simulink model "DC_control"  (R2023b)
settings: Solver=ode45  StartTime=0.0  StopTime=700  RelTol=1e-3
values from neighbouring files (symbols this model uses):
  g = 9.81    [Parameters_estimation.m]
  Ia_n = (Ptot-Ve_n*Ie_n)/Va_n    [Parameters_estimation.m]    (also in psi_ref_parameters.mat = 650.546469803)
  Ke = Pn/(Ie_n*Ia_n*w_n)    [Parameters_estimation.m]    (also in psi_ref_parameters.mat = 1.72027393081)
  M = 10*10^3+80*200    (= 26000)    [Parameters_estimation.m]
  mu_Ia = 1/Ra    [Parameters_estimation.m]
  mu_Ie = 1/Re    (= 0.00833333333333)    [Parameters_estimation.m]
  mu_m = 1/(R^2*betha)    [Parameters_estimation.m]
  R = v_n/w_n    (= 0.0530785562633)    [Parameters_estimation.m]    (also in Radius.mat; my_parameters.mat)
  T_n = Ft_n * R    [Parameters_estimation.m]
  tau_Ia = La/Ra    [Parameters_estimation.m]
  tau_Ie = Le/Re    (= 1)    [Parameters_estimation.m]
  tau_m = M/betha    [Parameters_estimation.m]
  Va_n = 600    [Parameters_estimation.m]    (also in psi_ref_parameters.mat)
  Ve_n = 120    [Parameters_estimation.m]
  wc_Ia = 100    [Parameters_estimation.m]
  wc_Ie = 10    [Parameters_estimation.m]
  wc_ome = 5/(t_fin-20)    (= 1)    [Parameters_estimation.m]
libraries: slpidlib x3
settings Model: Creator=lmarz  LastModifiedBy=lmarz

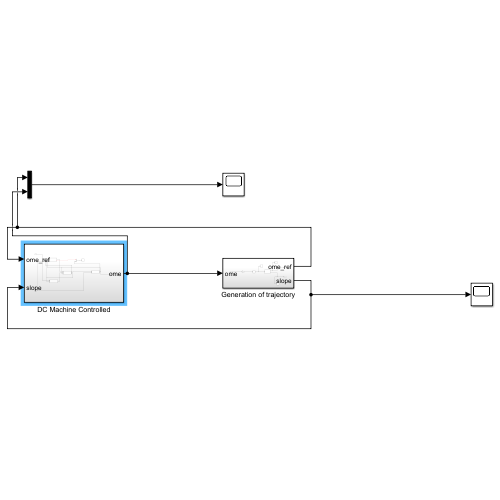
[thumbnail: Simulink's stored preview of the top-level diagram]
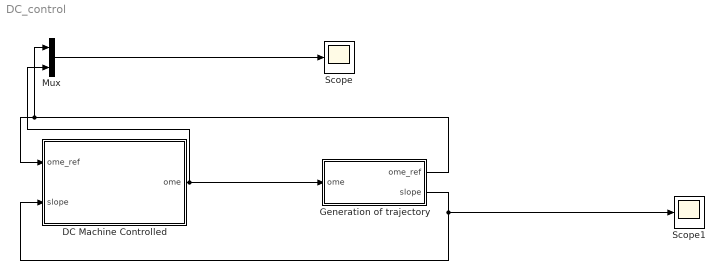
== system DC_control ==
  DC Machine Controlled : Subsystem
  Generation of trajectory : Subsystem
  Mux : Mux  Inputs=2
  Scope : Scope
  Scope1 : Scope
  wires:
  DC Machine Controlled/1(ome) -> Mux/2, Generation of trajectory/1(ome)
  Generation of trajectory/1(ome_ref) -> Mux/1, DC Machine Controlled/1(ome_ref)
  Generation of trajectory/2(slope) -> Scope1/1, DC Machine Controlled/2(slope)
  Mux/1 -> Scope/1

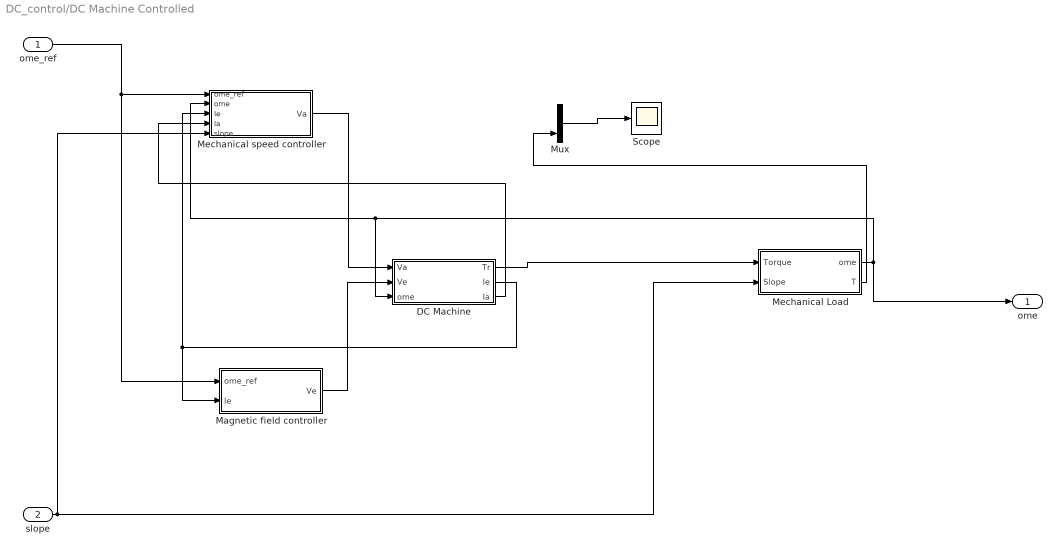
== system DC_control/DC Machine Controlled ==
  ome_ref : Inport
  slope : Inport  Port=2
  " Mechanical speed controller" : Subsystem
  DC Machine : Subsystem
  Magnetic field controller : Subsystem
  Mechanical Load : Subsystem
  Mux : Mux  Inputs=2
  Scope : Scope
  ome : Outport
  wires:
  DC Machine/1(Tr) -> Mechanical Load/1(Torque)
  Mechanical Load/1(ome) -> ome/1, DC Machine/3(ome), " Mechanical speed controller"/2(ome)
  ome_ref/1 -> Magnetic field controller/1(ome_ref), " Mechanical speed controller"/1(ome_ref)
  Magnetic field controller/1(Ve) -> DC Machine/2(Ve)
  DC Machine/2(Ie) -> " Mechanical speed controller"/3(Ie), Magnetic field controller/2(Ie)
  DC Machine/3(Ia) -> " Mechanical speed controller"/4(Ia)
  " Mechanical speed controller"/1(Va) -> DC Machine/1(Va)
  slope/1 -> " Mechanical speed controller"/5(slope), Mechanical Load/2(Slope)
  ? -> Mux/1
  Mechanical Load/2(T) -> Mux/2
  Mux/1 -> Scope/1

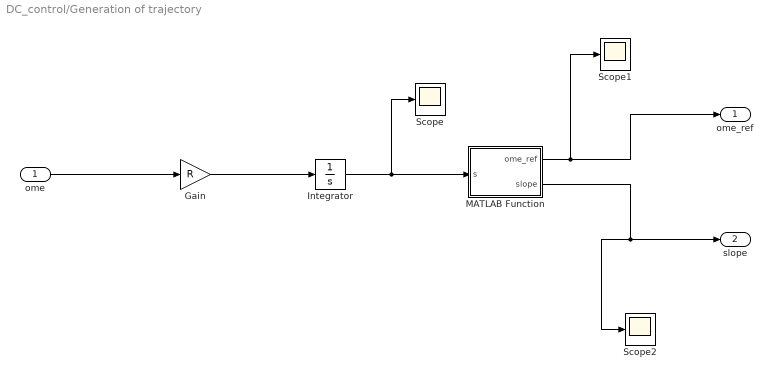
== system DC_control/Generation of trajectory ==
  ome : Inport
  Gain : Gain  Gain=R
  Integrator : Integrator
  MATLAB Function : MATLAB Function  TreatAsAtomicUnit=on
  Scope : Scope
  Scope1 : Scope
  Scope2 : Scope
  ome_ref : Outport
  slope : Outport  Port=2
  wires:
  ome/1 -> Gain/1
  Gain/1 -> Integrator/1
  Integrator/1 -> Scope/1, MATLAB Function/1(s)
  MATLAB Function/1(ome_ref) -> Scope1/1, ome_ref/1
  MATLAB Function/2(slope) -> Scope2/1, slope/1

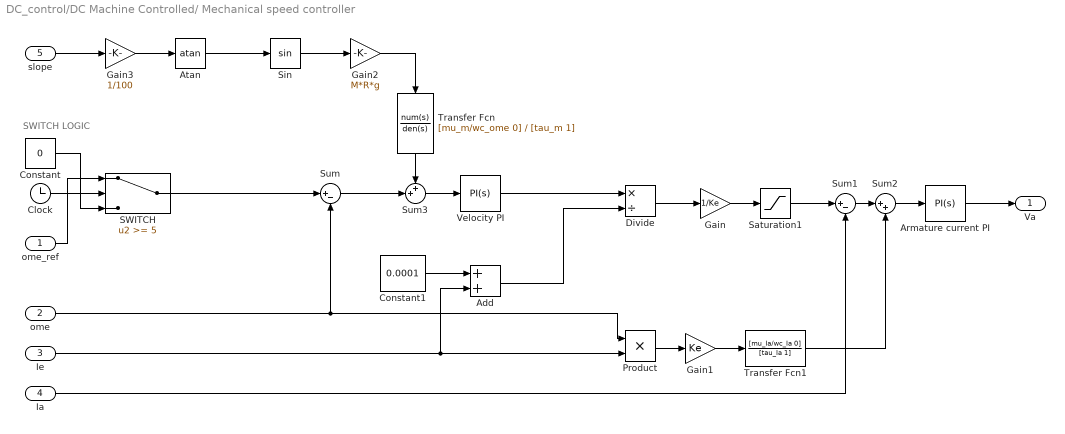
== system DC_control/DC Machine Controlled/ Mechanical speed controller ==
  note: SWITCH LOGIC
  ome_ref : Inport
  ome : Inport  Port=2
  Ie : Inport  Port=3
  Ia : Inport  Port=4
  slope : Inport  Port=5
  Add : Sum
  Armature current PI : slpidlib/PID Controller  Controller=PI  Form=Parallel  TimeDomain=Continuous-time  UseExternalTs=off  SampleTime=-1  IntegratorMethod=Forward Euler  FilterMethod=Forward Euler  ControllerParametersSource=internal  P=wc_Ia*tau_Ia/mu_Ia  I=wc_Ia/mu_Ia  UseKiTs=off  D=0  N=100  UseFilter=on  TunerSelectOption=Transfer Function Based (PID Tuner App)  ZeroCross=off  InitialConditionSource=internal  InitialConditionForIntegrator=0  InitialConditionForFilter=0  DifferentiatorICPrevScaledInput=0  ExternalReset=none  TrackingMode=off  Kt=1  LimitOutput=on  SatLimitsSource=internal  UpperSaturationLimit=Va_n  LowerSaturationLimit=-Va_n  LinearizeAsGain=on  AntiWindupMode=clamping  Kb=1  LimitIntegrator=off  UpperIntegratorSaturationLimit=inf  LowerIntegratorSaturationLimit=-inf  POutMin=[]  POutMax=[]  IOutMin=[]  IOutMax=[]  DOutMin=[]  DOutMax=[]  NOutMin=[]  NOutMax=[]  SumOutMin=[]  SumOutMax=[]  SaturationOutMin=[]  SaturationOutMax=[]  PParamMin=[]  PParamMax=[]  IParamMin=[]  IParamMax=[]  DParamMin=[]  DParamMax=[]  NParamMin=[]  NParamMax=[]  KbParamMin=[]  KbParamMax=[]  KtParamMin=[]  KtParamMax=[]  KbOutMin=[]  KbOutMax=[]  KtOutMin=[]  KtOutMax=[]  IntegratorOutMin=[]  IntegratorOutMax=[]  FilterOutMin=[]  FilterOutMax=[]  SumI1OutMin=[]  SumI1OutMax=[]  SumI2OutMin=[]  SumI2OutMax=[]  SumI3OutMin=[]  SumI3OutMax=[]  SumI4OutMin=[]  SumI4OutMax=[]  SumDOutMin=[]  SumDOutMax=[]  DifferentiatorOutMin=[]  DifferentiatorOutMax=[]  FilterDiffOutCoefMin=[]  FilterDiffOutCoefMax=[]  ReciprocalOutMin=[]  ReciprocalOutMax=[]  SumDenOutMin=[]  SumDenOutMax=[]  SumNumOutMin=[]  SumNumOutMax=[]  DivideOutMin=[]  DivideOutMax=[]  UdiffTsProdOutMin=[]  UdiffTsProdOutMax=[]  NTsProdOutMin=[]  NTsProdOutMax=[]  UintegralTsProdOutMin=[]  UintegralTsProdOutMax=[]  UngainTsProdOutMin=[]  UngainTsProdOutMax=[]  ClampingZeroOutDataTypeStr=Inherit: Inherit via back propagation  ClampingZeroOutMin=[]  ClampingZeroOutMax=[]  FilterDenConstantOutDataTypeStr=Inherit: Inherit via back propagation  FilterDenConstantOutMin=[]  FilterDenConstantOutMax=[]  PCopyOutDataTypeStr=Inherit: Inherit via back propagation  PCopyOutMin=[]  PCopyOutMax=[]  NCopyOutDataTypeStr=Inherit: Inherit via back propagation  NCopyOutMin=[]  NCopyOutMax=[]  IntegratorContinuousStateAttributes=''  IntegratorStateMustResolveToSignalObject=off  IntegratorRTWStateStorageClass=Auto  FilterContinuousStateAttributes=''  FilterStateMustResolveToSignalObject=off  FilterRTWStateStorageClass=Auto  ParallelPVariant=InternalParameters  IdealPVariant=Disabled  IVariant=InternalParameters  DVariant=Disabled  IntegratorVariant=Continuous  SatVariant=Enabled  AWVariant=ContClampingParallel  PCopyVariant=Disabled  TRVariant=Disabled  FdbkBlocksVariant=Forward  IdealPFdbkVariant=Disabled  SatFdbkVariant=Disabled  DerivativeFilterVariant=Disabled  NVariant=Disabled  NCopyVariant=Disabled_SignalSpec  FilterICVariant=Disabled  IntegratorICVariant=InternalICs  ExternalResetVariant=Disabled  TRSumVariant=Passthrough  SumFdbkVariant=Disabled  SumVariant=Sum_PI  TsampFilterVariant=InternalTs  TsampNgainVariant=Passthrough  TsampIntegralVariant=Disabled_SignalSpec  ExternalSaturationOutDataTypeStr=Inherit: Same as second input
  Atan : Trigonometry  Operator=atan
  Clock : Clock
  Constant : Constant  Value=0
  Constant1 : Constant  Value=0.0001
  Divide : Product  Inputs=*/
  Gain : Gain  Gain=1/Ke
  Gain1 : Gain  Gain=Ke
  Gain2 : Gain  Gain=M*R*g
  Gain3 : Gain  Gain=1/100
  Product : Product
  SWITCH : Switch  Threshold=5  SaturateOnIntegerOverflow=off  InputSameDT=off
  Saturation1 : Saturate  UpperLimit=Ia_n  LowerLimit=-Ia_n
  Sin : Trigonometry
  Sum : Sum  Inputs=|+-
  Sum1 : Sum  Inputs=|+-
  Sum2 : Sum  Inputs=|++
  Sum3 : Sum  Inputs=++|
  Transfer Fcn : TransferFcn  Numerator=[mu_m/wc_ome 0]  Denominator=[tau_m 1]
  Transfer Fcn1 : TransferFcn  Numerator=[mu_Ia/wc_Ia 0]  Denominator=[tau_Ia 1]
  Velocity PI : slpidlib/PID Controller  Controller=PI  Form=Parallel  TimeDomain=Continuous-time  UseExternalTs=off  SampleTime=-1  IntegratorMethod=Forward Euler  FilterMethod=Forward Euler  ControllerParametersSource=internal  P=wc_ome*tau_m/mu_m  I=wc_ome/mu_m  UseKiTs=off  D=0  N=100  UseFilter=on  TunerSelectOption=Transfer Function Based (PID Tuner App)  ZeroCross=off  InitialConditionSource=internal  InitialConditionForIntegrator=0  InitialConditionForFilter=0  DifferentiatorICPrevScaledInput=0  ExternalReset=none  TrackingMode=off  Kt=1  LimitOutput=on  SatLimitsSource=internal  UpperSaturationLimit=T_n  LowerSaturationLimit=-T_n  LinearizeAsGain=on  AntiWindupMode=clamping  Kb=1  LimitIntegrator=off  UpperIntegratorSaturationLimit=inf  LowerIntegratorSaturationLimit=-inf  POutMin=[]  POutMax=[]  IOutMin=[]  IOutMax=[]  DOutMin=[]  DOutMax=[]  NOutMin=[]  NOutMax=[]  SumOutMin=[]  SumOutMax=[]  SaturationOutMin=[]  SaturationOutMax=[]  PParamMin=[]  PParamMax=[]  IParamMin=[]  IParamMax=[]  DParamMin=[]  DParamMax=[]  NParamMin=[]  NParamMax=[]  KbParamMin=[]  KbParamMax=[]  KtParamMin=[]  KtParamMax=[]  KbOutMin=[]  KbOutMax=[]  KtOutMin=[]  KtOutMax=[]  IntegratorOutMin=[]  IntegratorOutMax=[]  FilterOutMin=[]  FilterOutMax=[]  SumI1OutMin=[]  SumI1OutMax=[]  SumI2OutMin=[]  SumI2OutMax=[]  SumI3OutMin=[]  SumI3OutMax=[]  SumI4OutMin=[]  SumI4OutMax=[]  SumDOutMin=[]  SumDOutMax=[]  DifferentiatorOutMin=[]  DifferentiatorOutMax=[]  FilterDiffOutCoefMin=[]  FilterDiffOutCoefMax=[]  ReciprocalOutMin=[]  ReciprocalOutMax=[]  SumDenOutMin=[]  SumDenOutMax=[]  SumNumOutMin=[]  SumNumOutMax=[]  DivideOutMin=[]  DivideOutMax=[]  UdiffTsProdOutMin=[]  UdiffTsProdOutMax=[]  NTsProdOutMin=[]  NTsProdOutMax=[]  UintegralTsProdOutMin=[]  UintegralTsProdOutMax=[]  UngainTsProdOutMin=[]  UngainTsProdOutMax=[]  ClampingZeroOutDataTypeStr=Inherit: Inherit via back propagation  ClampingZeroOutMin=[]  ClampingZeroOutMax=[]  FilterDenConstantOutDataTypeStr=Inherit: Inherit via back propagation  FilterDenConstantOutMin=[]  FilterDenConstantOutMax=[]  PCopyOutDataTypeStr=Inherit: Inherit via back propagation  PCopyOutMin=[]  PCopyOutMax=[]  NCopyOutDataTypeStr=Inherit: Inherit via back propagation  NCopyOutMin=[]  NCopyOutMax=[]  IntegratorContinuousStateAttributes=''  IntegratorStateMustResolveToSignalObject=off  IntegratorRTWStateStorageClass=Auto  FilterContinuousStateAttributes=''  FilterStateMustResolveToSignalObject=off  FilterRTWStateStorageClass=Auto  ParallelPVariant=InternalParameters  IdealPVariant=Disabled  IVariant=InternalParameters  DVariant=Disabled  IntegratorVariant=Continuous  SatVariant=Enabled  AWVariant=ContClampingParallel  PCopyVariant=Disabled  TRVariant=Disabled  FdbkBlocksVariant=Forward  IdealPFdbkVariant=Disabled  SatFdbkVariant=Disabled  DerivativeFilterVariant=Disabled  NVariant=Disabled  NCopyVariant=Disabled_SignalSpec  FilterICVariant=Disabled  IntegratorICVariant=InternalICs  ExternalResetVariant=Disabled  TRSumVariant=Passthrough  SumFdbkVariant=Disabled  SumVariant=Sum_PI  TsampFilterVariant=InternalTs  TsampNgainVariant=Passthrough  TsampIntegralVariant=Disabled_SignalSpec  ExternalSaturationOutDataTypeStr=Inherit: Same as second input
  Va : Outport
  wires:
  ome/1 -> Sum/2, Product/1
  Gain/1 -> Saturation1/1
  Ia/1 -> Sum1/2
  Product/1 -> Gain1/1
  Armature current PI/1 -> Va/1
  Velocity PI/1 -> Divide/1
  Sin/1 -> Gain2/1
  slope/1 -> Gain3/1
  Gain3/1 -> Atan/1
  Atan/1 -> Sin/1
  Clock/1 -> SWITCH/2
  SWITCH/1 -> Sum/1
  Constant/1 -> SWITCH/3
  ome_ref/1 -> SWITCH/1
  Gain2/1 -> Transfer Fcn/1
  Sum3/1 -> Velocity PI/1
  Sum/1 -> Sum3/2
  Gain1/1 -> Transfer Fcn1/1
  Sum1/1 -> Sum2/1
  Sum2/1 -> Armature current PI/1
  Ie/1 -> Add/2, Product/2
  Constant1/1 -> Add/1
  Add/1 -> Divide/2
  Transfer Fcn1/1 -> Sum2/2
  Saturation1/1 -> Sum1/1
  Divide/1 -> Gain/1
  Transfer Fcn/1 -> Sum3/1

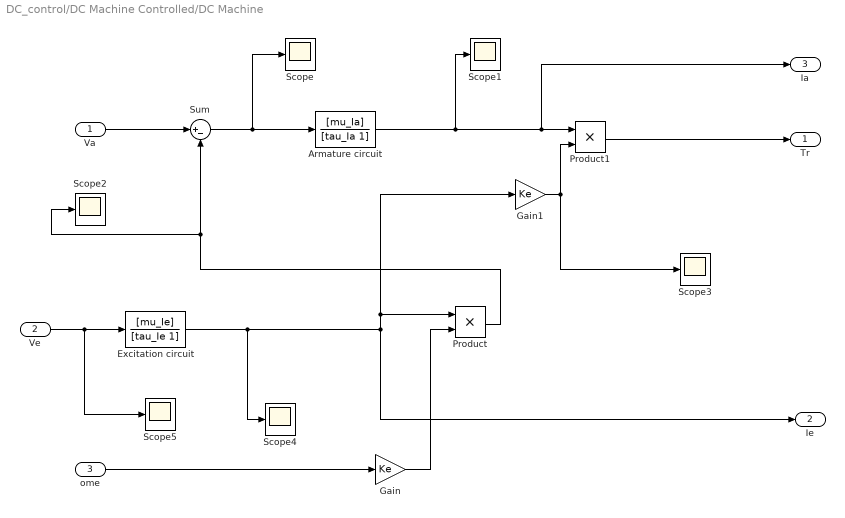
== system DC_control/DC Machine Controlled/DC Machine ==
  Va : Inport
  Ve : Inport  Port=2
  ome : Inport  Port=3
  Armature circuit : TransferFcn  Numerator=[mu_Ia]  Denominator=[tau_Ia 1]
  Excitation circuit : TransferFcn  Numerator=[mu_Ie]  Denominator=[tau_Ie 1]
  Gain : Gain  Gain=Ke
  Gain1 : Gain  Gain=Ke
  Product : Product
  Product1 : Product
  Scope{,1..5} (6 alike) : Scope
  Sum : Sum  Inputs=|+-
  Tr : Outport
  Ie : Outport  Port=2
  Ia : Outport  Port=3
  wires:
  Ve/1 -> Scope5/1, Excitation circuit/1
  Excitation circuit/1 -> Scope4/1, Ie/1, Product/1, Gain1/1
  Gain/1 -> Product/2
  Va/1 -> Sum/1
  Product/1 -> Sum/2, Scope2/1
  Sum/1 -> Scope/1, Armature circuit/1
  ome/1 -> Gain/1
  Armature circuit/1 -> Scope1/1, Ia/1, Product1/1
  Gain1/1 -> Product1/2, Scope3/1
  Product1/1 -> Tr/1

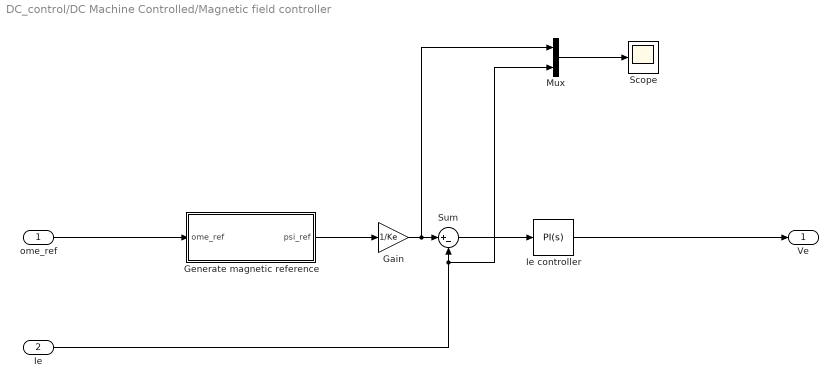
== system DC_control/DC Machine Controlled/Magnetic field controller ==
  ome_ref : Inport
  Ie : Inport  Port=2
  Gain : Gain  Gain=1/Ke
  Generate magnetic reference : MATLAB Function  TreatAsAtomicUnit=on
  Ie controller : slpidlib/PID Controller  Controller=PI  Form=Parallel  TimeDomain=Continuous-time  UseExternalTs=off  SampleTime=-1  IntegratorMethod=Forward Euler  FilterMethod=Forward Euler  ControllerParametersSource=internal  P=wc_Ie*tau_Ie/mu_Ie  I=wc_Ie/mu_Ie  UseKiTs=off  D=0  N=100  UseFilter=on  TunerSelectOption=Transfer Function Based (PID Tuner App)  ZeroCross=off  InitialConditionSource=internal  InitialConditionForIntegrator=0  InitialConditionForFilter=0  DifferentiatorICPrevScaledInput=0  ExternalReset=none  TrackingMode=off  Kt=1  LimitOutput=on  SatLimitsSource=internal  UpperSaturationLimit=Ve_n  LowerSaturationLimit=-Ve_n  LinearizeAsGain=on  AntiWindupMode=clamping  Kb=1  LimitIntegrator=off  UpperIntegratorSaturationLimit=inf  LowerIntegratorSaturationLimit=-inf  POutMin=[]  POutMax=[]  IOutMin=[]  IOutMax=[]  DOutMin=[]  DOutMax=[]  NOutMin=[]  NOutMax=[]  SumOutMin=[]  SumOutMax=[]  SaturationOutMin=[]  SaturationOutMax=[]  PParamMin=[]  PParamMax=[]  IParamMin=[]  IParamMax=[]  DParamMin=[]  DParamMax=[]  NParamMin=[]  NParamMax=[]  KbParamMin=[]  KbParamMax=[]  KtParamMin=[]  KtParamMax=[]  KbOutMin=[]  KbOutMax=[]  KtOutMin=[]  KtOutMax=[]  IntegratorOutMin=[]  IntegratorOutMax=[]  FilterOutMin=[]  FilterOutMax=[]  SumI1OutMin=[]  SumI1OutMax=[]  SumI2OutMin=[]  SumI2OutMax=[]  SumI3OutMin=[]  SumI3OutMax=[]  SumI4OutMin=[]  SumI4OutMax=[]  SumDOutMin=[]  SumDOutMax=[]  DifferentiatorOutMin=[]  DifferentiatorOutMax=[]  FilterDiffOutCoefMin=[]  FilterDiffOutCoefMax=[]  ReciprocalOutMin=[]  ReciprocalOutMax=[]  SumDenOutMin=[]  SumDenOutMax=[]  SumNumOutMin=[]  SumNumOutMax=[]  DivideOutMin=[]  DivideOutMax=[]  UdiffTsProdOutMin=[]  UdiffTsProdOutMax=[]  NTsProdOutMin=[]  NTsProdOutMax=[]  UintegralTsProdOutMin=[]  UintegralTsProdOutMax=[]  UngainTsProdOutMin=[]  UngainTsProdOutMax=[]  ClampingZeroOutDataTypeStr=Inherit: Inherit via back propagation  ClampingZeroOutMin=[]  ClampingZeroOutMax=[]  FilterDenConstantOutDataTypeStr=Inherit: Inherit via back propagation  FilterDenConstantOutMin=[]  FilterDenConstantOutMax=[]  PCopyOutDataTypeStr=Inherit: Inherit via back propagation  PCopyOutMin=[]  PCopyOutMax=[]  NCopyOutDataTypeStr=Inherit: Inherit via back propagation  NCopyOutMin=[]  NCopyOutMax=[]  IntegratorContinuousStateAttributes=''  IntegratorStateMustResolveToSignalObject=off  IntegratorRTWStateStorageClass=Auto  FilterContinuousStateAttributes=''  FilterStateMustResolveToSignalObject=off  FilterRTWStateStorageClass=Auto  ParallelPVariant=InternalParameters  IdealPVariant=Disabled  IVariant=InternalParameters  DVariant=Disabled  IntegratorVariant=Continuous  SatVariant=Enabled  AWVariant=ContClampingParallel  PCopyVariant=Disabled  TRVariant=Disabled  FdbkBlocksVariant=Forward  IdealPFdbkVariant=Disabled  SatFdbkVariant=Disabled  DerivativeFilterVariant=Disabled  NVariant=Disabled  NCopyVariant=Disabled_SignalSpec  FilterICVariant=Disabled  IntegratorICVariant=InternalICs  ExternalResetVariant=Disabled  TRSumVariant=Passthrough  SumFdbkVariant=Disabled  SumVariant=Sum_PI  TsampFilterVariant=InternalTs  TsampNgainVariant=Passthrough  TsampIntegralVariant=Disabled_SignalSpec  ExternalSaturationOutDataTypeStr=Inherit: Same as second input
  Mux : Mux  Inputs=2
  Scope : Scope
  Sum : Sum  Inputs=|+-
  Ve : Outport
  wires:
  ome_ref/1 -> Generate magnetic reference/1(ome_ref)
  Generate magnetic reference/1(psi_ref) -> Gain/1
  Gain/1 -> Mux/1, Sum/1
  Ie/1 -> Mux/2, Sum/2
  Sum/1 -> Ie controller/1
  Ie controller/1 -> Ve/1
  Mux/1 -> Scope/1

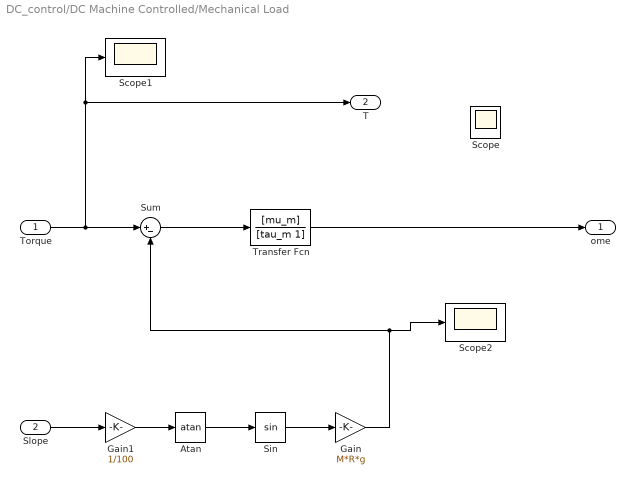
== system DC_control/DC Machine Controlled/Mechanical Load ==
  Torque : Inport
  Slope : Inport  Port=2
  Atan : Trigonometry  Operator=atan
  Gain : Gain  Gain=M*R*g
  Gain1 : Gain  Gain=1/100
  Scope : Scope
  Scope1 : Scope
  Scope2 : Scope
  Sin : Trigonometry
  Sum : Sum  Inputs=|+-
  Transfer Fcn : TransferFcn  Numerator=[mu_m]  Denominator=[tau_m 1]
  ome : Outport
  T : Outport  Port=2
  wires:
  Torque/1 -> T/1, Scope1/1, Sum/1
  Sum/1 -> Transfer Fcn/1
  Slope/1 -> Gain1/1
  Gain1/1 -> Atan/1
  Atan/1 -> Sin/1
  Sin/1 -> Gain/1
  Transfer Fcn/1 -> ome/1
  Gain/1 -> Scope2/1, Sum/2

== matlab function DC_control/DC Machine Controlled/Magnetic field controller/Generate magnetic reference ==
  data: ome_ref input; psi_ref output
function psi_ref = fcn(ome_ref)

par = load('psi_ref_parameters.mat');


if ome_ref < par.ome_b
    psi_ref = par.Ke*par.Ie_n;
else
    psi_ref = (par.Va_n-par.Ra*par.Ia_n)/ome_ref;
end

== matlab function DC_control/Generation of trajectory/MATLAB Function ==
  data: s input; ome_ref output; slope output
function [ome_ref, slope] = fcn(s)

a = load("radius.mat");
conv = 1000/3600/a.R;

if s >= 0 && s < 1000
    ome_ref = 35 * conv;
    slope = 0;
elseif s >= 1000 && s < 3000
    ome_ref = 60 * conv;
    slope = 0;
elseif s >= 3000 && s < 4000
    ome_ref = 60 * conv;
    slope = 5;
elseif s >= 4000 && s < 6000
    ome_ref = 75 * conv;
    slope = 0;
elseif s >= 6000 && s < 8000
    ome_ref = 60 * conv;
    slope = 0;
elseif s >= 8000 && s < 9000
    ome_ref = 60 * conv;
    slope = -5;
elseif s >= 9000
    ome_ref = 35 * conv;
    slope = 0;
else
    error('Value of s is out of expected range.');
end
